simulink model "sim_CS1B_nonlinear"  (R2025b)
settings: Solver=ode45  StartTime=0.0  StopTime=Tsim  MaxStep=ts  RelTol=1e-6
values from neighbouring files (symbols this model uses):
  a = a(k:end) / a(k)    [block_coeffs.m]    (also in qube_model.m = 0.000406791666667)
  b = b(k:end) / a(k)    [block_coeffs.m]    (also in qube_model.m = 0.000133128)
  c = mp*Lr*lp    (= 0.00013158)    [qube_model.m]
  d = Dr + kt*km/Rm    (= 0.00171)    [qube_model.m]
  Dp = 0.0005    [qube_model.m]
  h = mp*g*lp    (= 0.01518588)    [qube_model.m]
  kv = kt/Rm    (= 0.005)    [qube_model.m]
  step_time = 1    [design_and_simulate_CS1B.m]    (also in params_CS1B.m)
  theta_step = deg2rad(45)    [design_and_simulate_CS1B.m]    (also in params_CS1B.m = 0.785398163397)
  ts = 1/1000    (= 0.001)    [Hardware_settings.m]    (also in qube_model.m)
  x0 = zeros(4,1)    [design_and_simulate_CS1B.m]    (also in params_CS1B.m = [0; 0; 0; 0])
settings Model: Creator=jaylen  LastModifiedBy=jaylen
settings DataIOCC: SaveOutput=off  SaveTime=off
settings DebuggingCC: AlgebraicLoopMsg=none

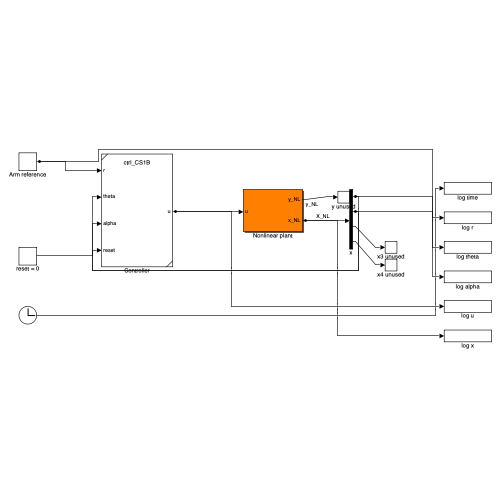
[thumbnail: Simulink's stored preview of the top-level diagram]
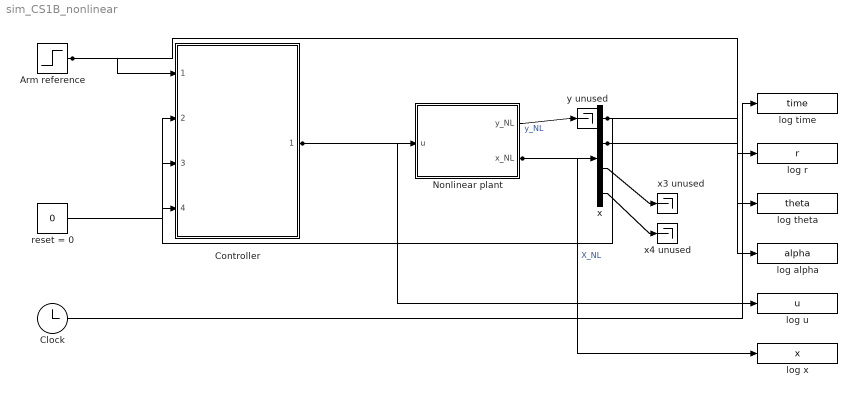
== system sim_CS1B_nonlinear ==
  Arm reference : Step  Time=step_time  After=theta_step  SampleTime=ts
  Clock : Clock
  Controller : Subsystem  ReferencedSubsystem=ctrl_CS1B
  Nonlinear plant : Subsystem
  log alpha : ToWorkspace  VariableName=alpha  SampleTime=ts
  log r : ToWorkspace  VariableName=r  SampleTime=ts
  log theta : ToWorkspace  VariableName=theta  SampleTime=ts
  log time : ToWorkspace  VariableName=time  SampleTime=ts
  log u : ToWorkspace  VariableName=u  SampleTime=ts
  log x : ToWorkspace  VariableName=x  SampleTime=ts
  reset = 0 : Constant  Value=0
  x : Demux
  x3 unused : Terminator
  x4 unused : Terminator
  y unused : Terminator
  wires:
  Nonlinear plant/1(y_NL) -> y unused/1  "y_NL"
  Nonlinear plant/2(x_NL) -> x/1, log x/1  "X_NL"
  Controller/1 -> Nonlinear plant/1(u), log u/1
  Arm reference/1 -> Controller/1, log r/1
  x/1 -> Controller/2, log theta/1
  x/2 -> Controller/3, log alpha/1
  reset = 0/1 -> Controller/4
  x/3 -> x3 unused/1
  x/4 -> x4 unused/1
  Clock/1 -> log time/1

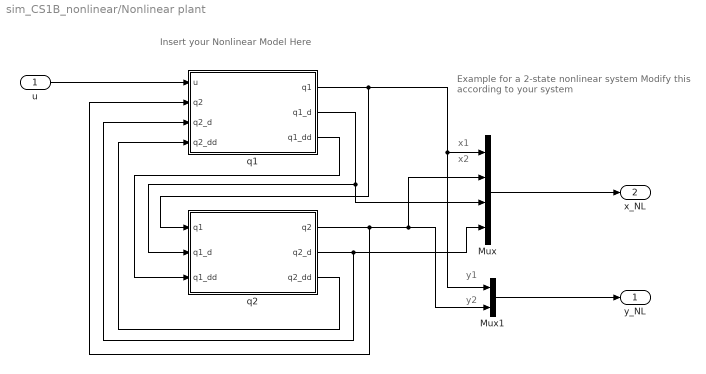
== system sim_CS1B_nonlinear/Nonlinear plant ==
  note: Example for a 2-state nonlinear system
      | Modify this according to your system
  note: y2
  note: y1
  note: x2
  note: Insert your Nonlinear Model Here
  note: x1
  u : Inport
  Mux : Mux
  Mux1 : Mux  Inputs=2
  q1 : Subsystem
  q2 : Subsystem
  y_NL : Outport  VectorParamsAs1DForOutWhenUnconnected=off
  x_NL : Outport  Port=2  VectorParamsAs1DForOutWhenUnconnected=off
  wires:
  q1/3(q1_dd) -> q2/3(q1_dd)
  u/1 -> q1/1(u)
  Mux1/1 -> y_NL/1
  Mux/1 -> x_NL/1
  q1/1(q1) -> Mux/1, Mux1/1, q2/1(q1)
  q1/2(q1_d) -> q2/2(q1_d), Mux/3
  q2/1(q2) -> q1/2(q2), Mux1/2, Mux/2
  q2/2(q2_d) -> q1/3(q2_d), Mux/4
  q2/3(q2_dd) -> q1/4(q2_dd)

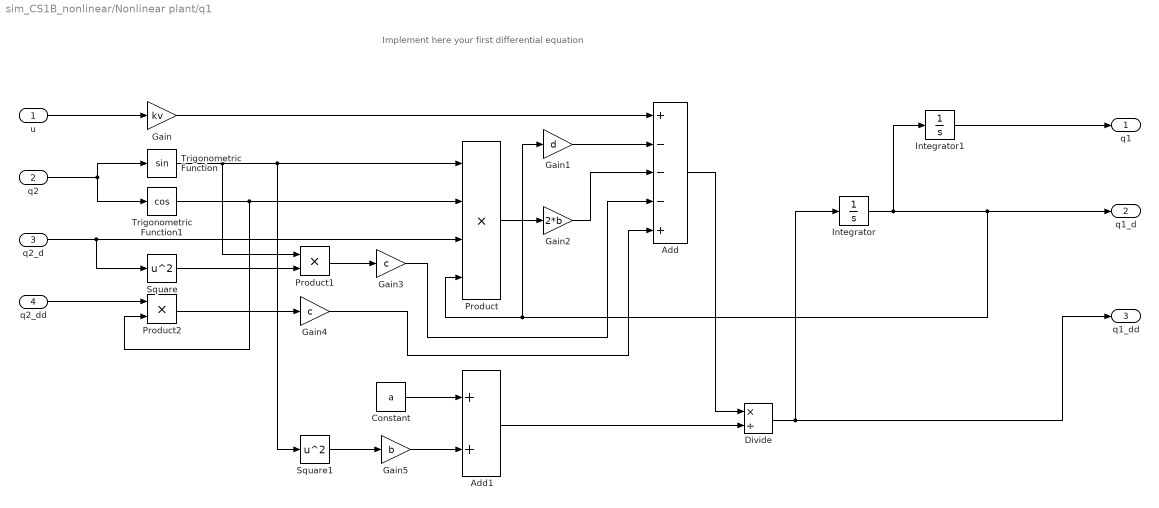
== system sim_CS1B_nonlinear/Nonlinear plant/q1 ==
  note: Implement here your first differential equation
  u : Inport
  q2 : Inport  Port=2
  q2_d : Inport  Port=3
  q2_dd : Inport  Port=4
  Add : Sum  Inputs=+---+
  Add1 : Sum
  Constant : Constant  Value=a
  Divide : Product  Inputs=*/
  Gain : Gain  Gain=kv
  Gain1 : Gain  Gain=d
  Gain2 : Gain  Gain=2*b
  Gain3 : Gain  Gain=c
  Gain4 : Gain  Gain=c
  Gain5 : Gain  Gain=b
  Integrator : Integrator  InitialCondition=x0(3)
  Integrator1 : Integrator  InitialCondition=x0(1)
  Product : Product  Inputs=4
  Product1 : Product
  Product2 : Product
  Square : Math  Operator=square
  Square1 : Math  Operator=square
  Trigonometric Function : Trigonometry
  Trigonometric Function1 : Trigonometry  Operator=cos
  q1 : Outport  VectorParamsAs1DForOutWhenUnconnected=off
  q1_d : Outport  Port=2  VectorParamsAs1DForOutWhenUnconnected=off
  q1_dd : Outport  Port=3  VectorParamsAs1DForOutWhenUnconnected=off
  wires:
  Constant/1 -> Add1/1
  Gain5/1 -> Add1/2
  Gain1/1 -> Add/2
  Divide/1 -> q1_dd/1, Integrator/1
  Add1/1 -> Divide/2
  Add/1 -> Divide/1
  Square1/1 -> Gain5/1
  Gain4/1 -> Add/5
  Gain3/1 -> Add/4
  Gain2/1 -> Add/3
  Gain/1 -> Add/1
  Product2/1 -> Gain4/1
  q2_dd/1 -> Product2/1
  Product1/1 -> Gain3/1
  Square/1 -> Product1/2
  Product/1 -> Gain2/1
  q2_d/1 -> Product/3, Square/1
  Trigonometric Function1/1 -> Product/2, Product2/2
  Trigonometric Function/1 -> Product1/1, Square1/1, Product/1
  q2/1 -> Trigonometric Function/1, Trigonometric Function1/1
  u/1 -> Gain/1
  Integrator1/1 -> q1/1
  Integrator/1 -> Integrator1/1, q1_d/1, Product/4, Gain1/1

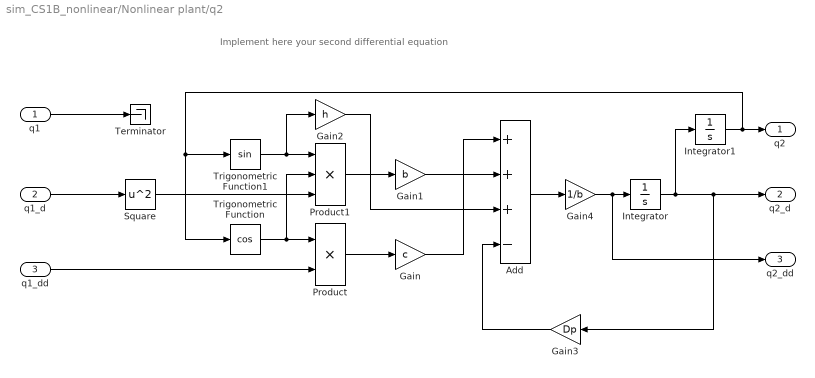
== system sim_CS1B_nonlinear/Nonlinear plant/q2 ==
  note: Implement here your second differential equation
  q1 : Inport
  q1_d : Inport  Port=2
  q1_dd : Inport  Port=3
  Add : Sum  Inputs=+++-
  Gain : Gain  Gain=c
  Gain1 : Gain  Gain=b
  Gain2 : Gain  Gain=h
  Gain3 : Gain  Gain=Dp
  Gain4 : Gain  Gain=1/b
  Integrator : Integrator  InitialCondition=x0(4)
  Integrator1 : Integrator  InitialCondition=x0(2)
  Product : Product
  Product1 : Product  Inputs=3
  Square : Math  Operator=square
  Terminator : Terminator
  Trigonometric Function : Trigonometry  Operator=cos
  Trigonometric Function1 : Trigonometry
  q2 : Outport  VectorParamsAs1DForOutWhenUnconnected=off
  q2_d : Outport  Port=2  VectorParamsAs1DForOutWhenUnconnected=off
  q2_dd : Outport  Port=3  VectorParamsAs1DForOutWhenUnconnected=off
  wires:
  Gain4/1 -> Integrator/1, q2_dd/1
  Add/1 -> Gain4/1
  Gain3/1 -> Add/4
  Gain2/1 -> Add/3
  Gain1/1 -> Add/2
  Gain/1 -> Add/1
  Square/1 -> Product1/3
  Product1/1 -> Gain1/1
  Trigonometric Function1/1 -> Product1/1, Gain2/1
  q1_d/1 -> Square/1
  Product/1 -> Gain/1
  Trigonometric Function/1 -> Product/1, Product1/2
  q1_dd/1 -> Product/2
  q1/1 -> Terminator/1
  Integrator1/1 -> q2/1, Trigonometric Function/1, Trigonometric Function1/1
  Integrator/1 -> q2_d/1, Gain3/1, Integrator1/1
